simulink model "hrg_bias_tdm_separate"  (R2025a)
settings: Solver=FixedStepDiscrete  StartTime=0.0  StopTime=(floor(c.duration/L.T+1e-9)-1)*L.T  FixedStep=L.T  RelTol=1e-3
model workspace (MAT data in the model file):
  L.F = [0.999580876972 3.24694996317e-07 6.81989764392e-05 6.22779391701e-05 5.91705719226e-22 1.19137426687e-24 -3.75693094649e-06 -6.22765091713e-07 0.0307885035579 6.20769031032e-05 0 0 ... (676 elements, 26x26)]
  L.G = [-0.000337166724513  -2.04304384739e-07  -0.00375589625801  5.33282123475e-09; -2.04543780755e-07  -0.000336718961012  3.19516910592e-09  -0.00375590559772; 0.00375588661538  -2.39457733197e-08  -0.000337166687299  -2.0423130018e-07; -2.18248235755e-08  0.00375593674255  -2.04470629604e-07  -0.000336719083954; 2.59647192694e-23  -2.85679187492e-28  -4.5702926148e-24  -1.40870743879e-27; -7.50589339501e-28  7.17545438659e-23  -3.90090208289e-27  -1.26447354992e-23; -3.75578257448e-05  2.40080747261e-10  3.383220588e-06  2.0422391658e-09; 2.18872587298e-10  -3.75583283826e-05  2.04463898185e-09  3.37874470913e-06; 0.00374197693059  -3.01302631226e-08  -0.000452279130212  -2.03304674872e-07; -2.80246387116e-08  0.00374204062084  -2.03608755041e-07  -0.000451833485601; 0  0  0  0; 0  0  0  0; -0.00154586308247  -1.73922924704e-07  -0.00321638953928  7.06995124769e-08; -1.74820024684e-07  -0.00154548114517  6.88761221884e-08  -0.00321654240012; 0  0  0  0; 0  0  0  0; -0.00236595352656  -1.3071982655e-07  -0.00241196525268  1.1512833246e-07; -1.32042498131e-07  -0.00236566575377  1.13754487179e-07  -0.00241221592121; 0  0  0  0; 0  0  0  0; -0.0028559083186  -7.99186721916e-08  -0.00144095630782  1.42291193957e-07; -8.1478017053e-08  -0.00285573155971  1.414473285e-07  -0.00144126705338; 0  0  0  0; 0  0  0  0; -0.00299916333611  -2.7641740102e-08  -0.000421240643113  1.51686649037e-07; -2.92493876018e-08  -0.00299910102992  1.51389176194e-07  -0.000421572566559]
  L.Hm = [0.999684417191  -1.48369934019e-06  -4.27964442652e-05  -4.66872440298e-05  -8.76929181689e-06  -4.76033457184e-09  -2.77456675998e-15  -3.69759326305e-16  2.43670473864e-11  3.69053916892e-14  0  0  0  0  0  0  0  0  0  0  0  0  0  0  0  0; -9.95250815563e-07  0.999687132089  -4.67001934864e-05  5.94798760013e-05  -4.76590244423e-09  -8.75885884545e-06  -3.69863076005e-16  -1.96454498714e-15  3.69274884564e-14  2.4286186882e-11  0  0  0  0  0  0  0  0  0  0  0  0  0  0  0  0; 7.61663704353e-05  4.67327413513e-05  0.999689714407  3.47258972194e-06  0.000102201297366  -5.08100401249e-11  7.91754167661e-12  2.73891160432e-17  -7.91004583605e-10  -1.61451620118e-15  0  0  0  0  0  0  0  0  0  0  0  0  0  0  0  0; 4.66938598472e-05  -2.61528408374e-05  3.96124178836e-06  0.999681573002  -9.63729064099e-13  0.000102201354068  3.12592084879e-17  7.91747744597e-12  -2.0008486826e-15  -7.91000624119e-10  0  0  0  0  0  0  0  0  0  0  0  0  0  0  0  0]
  L.Jm = [-0.000337106170818  -1.45329445201e-07  -0.00375629387149  4.42303169643e-09; -1.4556259223e-07  -0.000336787590847  2.90233098369e-09  -0.0037563018941; 0.00375629287294  -4.43692118232e-09  -0.000337233307174  -1.47097873108e-07; -2.91469077935e-09  0.0037563009243  -1.47136257932e-07  -0.000336911066999]
  L.Hc = [0.999712525524  1.91858120311e-06  -6.15968747997e-05  -4.30791897988e-05  -8.77146029918e-06  -4.42130011438e-09  -2.92353463991e-15  -3.41191828511e-16  2.43826074769e-11  3.41333263065e-14  0  0  -1.05090176987e-17  0  0  0  -6.61884364746e-19  0  0  0  -2.78073123766e-20  0  0  0  -5.84450076089e-22  0; 2.36910188548e-06  0.999707829722  -4.30567486948e-05  3.27377280262e-05  -4.4229173289e-09  -8.76177426388e-06  -3.41015192585e-16  -2.17639320848e-15  3.41264969975e-14  2.43078504888e-11  0  0  0  -1.05090176987e-17  0  0  0  -6.61884364746e-19  0  0  0  -2.78073123766e-20  0  0  0  -5.84450076089e-22; 6.4439329659e-05  4.41588003056e-05  0.999705540775  2.16132091986e-06  0.000102203018173  -1.62298309029e-10  7.91766705e-12  1.7010139137e-17  -7.91017391745e-10  -6.39624237198e-16  0  0  1.62851688606e-17  0  0  0  1.04154327129e-18  0  0  0  4.44136721082e-20  0  0  0  9.47053371996e-22  0; 4.41337760248e-05  -3.22571857823e-05  2.62312072719e-06  0.999700300936  -1.15318707191e-10  0.000102203322214  2.06675279441e-17  7.91762578606e-12  -1.00437249736e-15  -7.91015591268e-10  0  0  0  1.62851688606e-17  0  0  0  1.04154327129e-18  0  0  0  4.44136721082e-20  0  0  0  9.47053371996e-22]
  L.Jc = [-0.000337186287065  -1.32918322919e-07  -0.0037563931516  -9.57826075507e-09; -1.33005698555e-07  -0.000336895051636  -1.0968370094e-08  -0.00375637064928; 0.00375635629289  -8.4966552311e-09  -0.000337194577217  -1.36983680769e-07; -7.07999835389e-09  0.00375637335218  -1.37065085409e-07  -0.000336894443708]
  L.T = 0.000588235294118
  L.cvMap = [0.1458556769 -1.25015829619e-05 0.150764764274 -1.24845611429e-05 0.155664550533 -1.24667221104e-05 0.160554733441 -1.24480654683e-05 0.165435011352 -1.24285908741e-05 0.170305083231 -1.24082980387e-05 ... (96000 elements, 3200x30)]
  L.candidateOffset_s = 0.000515625
  biasWeights = [2.25592531536e-13; -5.76887878015e-06; 6.31924199918e-06; -0.00170881215954; 0.000155581549194]
  c.mode = 'tdm_separate'
  c.reuse = 0
  c.continuous = 0
  c.Ts = 1.83823529412e-07
  c.w = 42725.6600888
  c.omega = -0.001
  c.duration = 20
  c.B = 0.276990961962
  c.n = 800
  c.adcLatency = 5
  c.logDecimation = 200
  c.p.schema = 'v10.1'
  c.p.synthetic = 1
  c.p.f0 = 6800
  c.p.gamma_intrinsic = 0.712094334814
  c.p.Cs = 7.2e-10
  c.p.G0 = 1e-10
  c.p.kappa = 1e-06
  c.p.b = 1.1e-06
  c.p.Cds = 0
  c.p.Rs = 1000
  c.p.B = 0.276990961962
  c.p.Omega = -0.001
  c.p.Ts = 1.83823529412e-07
  c.p.Tc = 0.001
  c.p.duration = 20
  c.p.charge_target = 1e-11
  c.p.initial_fraction = 1
  c.p.theta0 = 0.981747704247
  c.p.Cf = 1e-10
  c.p.Rf = 1000000000
  c.p.driver_tau = [2e-06; 2e-06]
  c.p.afe_bw = [20000; 20000]
  c.p.detect_matrix = [1  0; 0  1]
  c.p.drive_matrix = [20  0; 0  20]
  c.p.split_hz = 0.05
  c.p.stiffness_axis = 0.37
  c.p.damping_half_difference = 0
  c.p.damping_axis = -0.23
  c.p.adc_span = 2
  c.p.adc_bits = 40
  c.p.dac_span = 1
  c.p.dac_bits = 40
  c.p.vmax = 0.5
  c.p.agc_bw = 10
  c.p.quad_bw = 4
  c.p.pll_gain = 30
  c.p.max_detune = 30
  c.p.virtual_rate = 0
  c.p.virtual_start_min_s = 0.25
  c.p.virtual_settle_fraction = 0.01
  c.p.predict_heading = 1
  c.p.max_heading_rate = 100
  c.p.virtual_validated_limit = 0.2
  c.p.min_amplitude_fraction = 0.02
  c.p.min_linearity = 0.1
  c.p.max_calibration_condition = 100
  c.p.max_frame_age = 0.002
  c.p.calibrate_detection = 1
  c.p.calibrate_drive = 1
  c.p.noise_rms_V = 0
  c.p.noise_seed = 52
  c.p.carrier_hz = 6800
  c.p.Q = 30000
  c.p.pre_gain = 1
  c.p.power_gain = 20
  c.p.aaf_order = 4
  c.p.fs = 5440000
  c.p.bleed_R = 2777.77854938
  c.p.reset_tau = 2e-06
  c.p.adc_latency = 5
  c.p.log_decimation = 200
  c.p.adc_noise_rms = 0
  c.p.adc_dither_lsb_rms = 0
  c.p.adc_dither_seeds = [1103515245; 2246822519]
  c.p.dac_divisor = 1
  c.p.allow_adc_underclock = 0
  c.p.seed_enabled = 0
  c.p.seed_seconds = 0.03
  c.p.seed_voltage = 0.2
  c.p.cv_mode = 'thx2024'
  c.p.thx_cv_gain = 10000
  c.p.thx_charge_per_input = 1e-06
  c.p.cv_source = 'thx2024'
  c.head.f0_Hz = 6800
  c.head.split_Hz = 0.05
  c.head.Q = 30000
  c.head.parasitic_F = 7.2e-10
  c.head.f_modes_Hz = [6799.975 6800.025]
  c.head.ringdown_s = 1.4043083214
  c.head.linewidth_Hz = 0.226666666667
  c.head.temperature_model = 'No per-head temperature curve supplied'
  c.head.group_shunt_F = [7.2e-10; 7.2e-10; 7.2e-10; 7.2e-10]
  c.driveEnd = 800
  c.senseStart = 1200
  c.validStart = 2000
  c.validEnd = 2800
  c.frame = 3200
  c.adcStep = 1.81898940355e-12
  c.adcMin = -1
  c.adcMax = 0.999999999998
  c.dacStep = 9.09494701773e-13
  c.dacMin = -0.5
  c.dacMax = 0.499999999999
  c.minEnergy = 0.0004
  c.minLinearity = 0.1
  c.agc = 62.8318530718
  c.gamma = 0.712094334814
  c.quad = 25.1327412287
  c.forceScale = 3.10732073373
  c.startCommand = [0; 0; 0; 0]
  c.seedCommand = [0; 0; -0.111114046604; -0.166293922461]
  c.stateCount = 26
  c.pickoff = [0  0  0  0  0  0  0  0  0  0  0  0  0  0  0  0  0  0  0  0  0  0  0  0  -0.8  0; 0  0  0  0  0  0  0  0  0  0  0  0  0  0  0  0  0  0  0  0  0  0  0  0  0  -0.8]
  c.motion = [1  0  0  0  0  0  0  0  0  0  0  0  0  0  0  0  0  0  0  0  0  0  0  0  0  0; 0  1  0  0  0  0  0  0  0  0  0  0  0  0  0  0  0  0  0  0  0  0  0  0  0  0]
  c.electrode = [0  0  0  0  0  0  0  0  -0.000427256600888  0  0  0  0  0  0  0  0  0  0  0  0  0  0  0  0  0; 0  0  0  0  0  0  0  0  0  -0.000427256600888  0  0  0  0  0  0  0  0  0  0  0  0  0  0  0  0]
  c.cvOutputGain = 10000
  c.Ad = [0.999969157815 1.52913483819e-10 -0.0078538572151 3.89384302746e-08 -2.77791419972e-24 3.37636119045e-29 7.54624297663e-05 -3.74133744973e-10 -0.000922446324141 4.57342487404e-09 0 0 ... (676 elements, 26x26)]
  c.Bd = [9.92930166753e-10  -3.47455020638e-20; 6.32815022009e-20  9.92930166722e-10; 3.90624565077e-07  -1.63776477948e-17; 3.51196242248e-17  3.90624565057e-07; 0.0878143670381  -3.30600504134e-39; 1.4384601036e-38  0.0878143670381; 3956.34070317  1.48469609002e-19; -3.08984060094e-19  3956.34070317; 3.03749598347e-08  -1.07224009297e-18; 1.96290342016e-18  3.03749598337e-08; 0  0; 0  0; 2.63190636606e-13  -6.89445846608e-24; 1.05402170351e-23  2.63190636602e-13; 0  0; 0  0; 9.85537732628e-16  -2.28470915408e-26; 3.30795441844e-26  9.85537732617e-16; 0  0; 0  0; 3.16265867511e-18  -6.57380608771e-29; 9.12786227069e-29  3.16265867508e-18; 0  0; 0  0; 8.88208109573e-21  -1.67304894509e-31; 2.24711851914e-31  8.88208109567e-21]
  c.Af = [0.999969157815 1.52913483819e-10 -0.0078538572151 3.89384302746e-08 -2.77791419972e-24 3.37636119045e-29 7.54624297663e-05 -3.74133744973e-10 -0.000922446324141 4.57342487404e-09 0 0 ... (676 elements, 26x26)]
  c.As = [0.999969157815 1.52913483819e-10 -0.0078538572151 3.89384302746e-08 -2.77791419972e-24 3.37636119045e-29 7.54624297663e-05 -3.74133744973e-10 -0.000922446324141 4.57342487404e-09 0 0 ... (676 elements, 26x26)]
  c.x0 = [0.55557023302; 0.831469612303; 0; 0; 0; 0; 0; 0; 0; 0; 0; 0; 0; 0; 0; 0; 0; 0; 0; 0; 0; 0; 0; 0; 0; 0]
  c.detect = [-0.353453438315  0  -1.51577588934  0; 0  -0.353453438315  0  -1.51577588934; 1.51577588934  0  -0.353453438315  0; 0  1.51577588934  0  -0.353453438315]
  c.drive = [0.049981589959  0  0.00448426958854  0; 0  0.049981589959  0  0.00448426958854; -0.00448426958854  0  0.049981589959  0; 0  -0.00448426958854  0  0.049981589959]
  c.gain_check.drive_pre_V_per_V = 1
  c.gain_check.sense_pre_V_per_V = 1
  c.gain_check.driver_post_gain = 20
  c.gain_check.detector_V_per_normalized_charge = 0.642491786495
  c.gain_check.electrode_limit_V = 10
  c.gain_check.drive_modal_V_per_command = 19.9273260068
  c.gain_check.drive_condition = 1
  c.gain_check.sense_condition = 1
  c.thx_comparison.saved_Kcvd = 10000
  c.thx_comparison.saved_Kcvs = 100000
  c.thx_comparison.saved_Kcsd = 10000
  c.thx_comparison.saved_Kcss = 100000
  c.thx_comparison.matched_cv_gain = 10000
  c.thx_comparison.piezo_charge_per_input_unit_C = 1e-06
  c.thx_comparison.reuse_scope = 'THX static readout Gain, matched to drive channel source value. Piezo adapter and AAF are external.'
  c.stateRows = {'1:4', '5:6', '7:10', '11:26'}
  c.portDriveMap = [1  0; 0  1; 0  0; 0  0]
  c.portSenseMap = [0  0  -8  0; 0  0  0  -8]
  c.portCoupling = [1  0; 0  1; -1  0; 0  -1]
  c.portCapacitance_F = [7.2e-10  0  0  0; 0  7.2e-10  0  0; 0  0  7.2e-10  0; 0  0  0  7.2e-10]
  c.portShuntCapacitance_F = [7.2e-10; 7.2e-10; 7.2e-10; 7.2e-10]
  c.groupAngles_deg = [0; 45; 90; 135]
  c.groupNames = {'A', 'B', 'C', 'D'}
  c.commonTerminal = 'COM'
  c.portOptions.group_angles_deg = [0; 45; 90; 135]
  c.portOptions.group_charge_gain = [1; 1; 1; 1]
  c.portOptions.group_capacitance_F = [7.2e-10; 7.2e-10; 7.2e-10; 7.2e-10]
  c.portOptions.drive_on_resistance_ohm = 10
  c.portOptions.diagnostic_carrier_phase_rad = []
  c.portCV = [0  0  0  0  0  0  0  0  0  0  0  0  0  0  0  0  0  0  0  0  0  0  0.1  0  0  0; 0  0  0  0  0  0  0  0  0  0  0  0  0  0  0  0  0  0  0  0  0  0  0  0.1  0  0; 0  0  0  0  0  0  0  0  0  0  0  0  0  0  0  0  0  0  0  0  0  0  0  0  0.1  0; 0  0  0  0  0  0  0  0  0  0  0  0  0  0  0  0  0  0  0  0  0  0  0  0  0  0.1]
  c.groupVoltage = [0  0  0  0  0  0  0.000427256600888  0  0  0  0  0  0  0  0  0  0  0  0  0  0  0  0  0  0  0; 0  0  0  0  0  0  0  0.000427256600888  0  0  0  0  0  0  0  0  0  0  0  0  0  0  0  0  0  0; 0  0  0  0  0  0  0  0  0.000427256600888  0  0  0  0  0  0  0  0  0  0  0  0  0  0  0  0  0; 0  0  0  0  0  0  0  0  0  0.000427256600888  0  0  0  0  0  0  0  0  0  0  0  0  0  0  0  0]
  c.periodicCarrier = 1
settings Model: Creator=Administrator  LastModifiedBy=Administrator

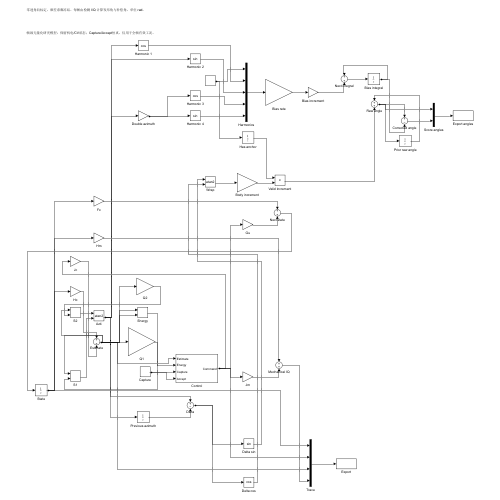
[thumbnail: Simulink's stored preview of the top-level diagram]
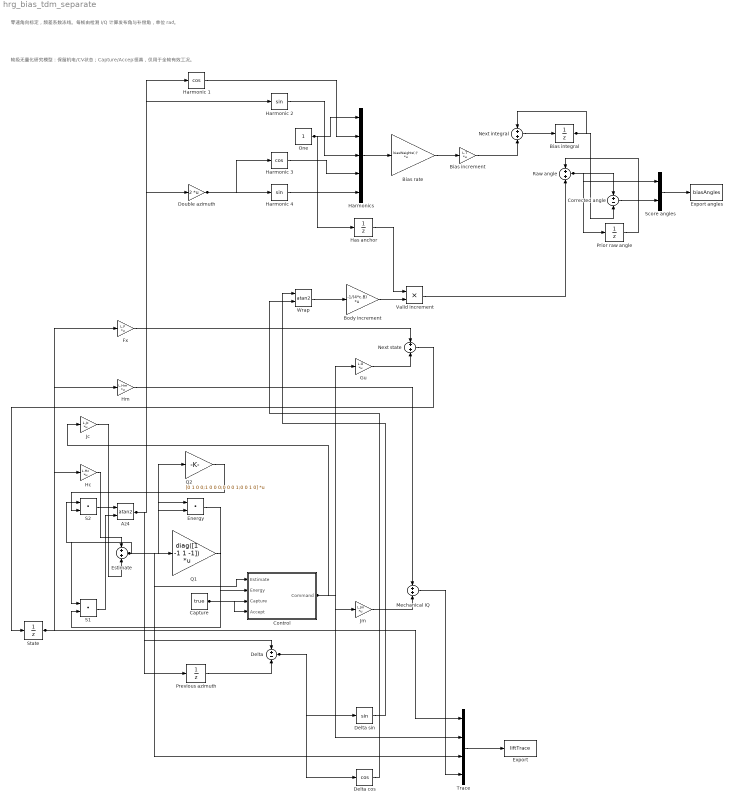
== system hrg_bias_tdm_separate ==
  note: 帧级无量化研究模型：保留机电/CV状态；Capture/Accept恒真，仅用于全帧有效工况。
  note: 零速角向标定，频差系数冻结。每帧由检测 I/Q 计算发布角与补偿角，单位 rad。
  Az4 : Trigonometry  Operator=atan2
  Bias increment : Gain  Gain=L.T  Multiplication=Matrix(K*u)
  Bias integral : UnitDelay  SampleTime=L.T  HasFrameUpgradeWarning=on
  Bias rate : Gain  Gain=biasWeights(:)'  Multiplication=Matrix(K*u)
  Body increment : Gain  Gain=-1/(4*c.B)  Multiplication=Matrix(K*u)
  Capture : Constant  Value=true  OutDataTypeStr=boolean
  Control : Subsystem
  Corrected angle : Sum  Inputs=+-
  Delta : Sum  Inputs=+-
  Delta cos : Trigonometry  Operator=cos
  Delta sin : Trigonometry
  Double azimuth : Gain  Gain=2  Multiplication=Matrix(K*u)
  Energy : DotProduct  OutDataTypeStr=Inherit: Inherit via internal rule
  Estimate : Sum
  Export : ToWorkspace  VariableName=liftTrace  SampleTime=-1
  Export angles : ToWorkspace  VariableName=biasAngles  SampleTime=-1
  Fx : Gain  Gain=L.F  Multiplication=Matrix(K*u)
  Gu : Gain  Gain=L.G  Multiplication=Matrix(K*u)
  Harmonic 1 : Trigonometry  Operator=cos
  Harmonic 2 : Trigonometry
  Harmonic 3 : Trigonometry  Operator=cos
  Harmonic 4 : Trigonometry
  Harmonics : Mux  Inputs=5
  Has anchor : UnitDelay  SampleTime=L.T  HasFrameUpgradeWarning=on
  Hc : Gain  Gain=L.Hc  Multiplication=Matrix(K*u)
  Hm : Gain  Gain=L.Hm  Multiplication=Matrix(K*u)
  Jc : Gain  Gain=L.Jc  Multiplication=Matrix(K*u)
  Jm : Gain  Gain=L.Jm  Multiplication=Matrix(K*u)
  Mechanical IQ : Sum
  Next integral : Sum
  Next state : Sum
  One : Constant
  Previous azimuth : UnitDelay  SampleTime=L.T  HasFrameUpgradeWarning=on
  Prior raw angle : UnitDelay  SampleTime=L.T  HasFrameUpgradeWarning=on
  Q1 : Gain  Gain=diag([1 -1 1 -1])  Multiplication=Matrix(K*u)
  Q2 : Gain  Gain=[0 1 0 0;1 0 0 0;0 0 0 1;0 0 1 0]  Multiplication=Matrix(K*u)
  Raw angle : Sum
  S1 : DotProduct  OutDataTypeStr=Inherit: Inherit via internal rule
  S2 : DotProduct  OutDataTypeStr=Inherit: Inherit via internal rule
  Score angles : Mux  Inputs=2
  State : UnitDelay  InitialCondition=c.x0  SampleTime=-1  HasFrameUpgradeWarning=on
  Trace : Mux
  Valid increment : Product
  Wrap : Trigonometry  Operator=atan2
  wires:
  Score angles/1 -> Export angles/1
  Corrected angle/1 -> Score angles/2
  Control/1(Command) -> Jc/1, Trace/2, Gu/1, Jm/1
  Hm/1 -> Mechanical IQ/1
  Hc/1 -> Estimate/1
  Jc/1 -> Estimate/2
  State/1 -> Fx/1, Hm/1, Hc/1, Trace/1
  S1/1 -> Az4/2
  Az4/1 -> Harmonic 2/1, Double azimuth/1, Harmonic 1/1, Previous azimuth/1, Delta/1
  S2/1 -> Az4/1
  Raw angle/1 -> Corrected angle/1, Score angles/1, Prior raw angle/1
  Energy/1 -> Control/2(Energy)
  Fx/1 -> Next state/1
  Prior raw angle/1 -> Raw angle/1
  Estimate/1 -> Control/1(Estimate), Energy/1, Q1/1, Q2/1, Trace/3, S1/1, Energy/2, S2/1
  Harmonic 1/1 -> Harmonics/2
  Double azimuth/1 -> Harmonic 4/1, Harmonic 3/1
  Q2/1 -> S2/2
  Q1/1 -> S1/2
  Capture/1 -> Control/4(Accept), Control/3(Capture)
  Wrap/1 -> Body increment/1
  Previous azimuth/1 -> Delta/2
  Bias rate/1 -> Bias increment/1
  Harmonic 2/1 -> Harmonics/3
  Harmonics/1 -> Bias rate/1
  One/1 -> Harmonics/1, Has anchor/1
  Harmonic 3/1 -> Harmonics/4
  Harmonic 4/1 -> Harmonics/5
  Delta cos/1 -> Wrap/2
  Delta/1 -> Delta sin/1, Delta cos/1
  Has anchor/1 -> Valid increment/1
  Body increment/1 -> Valid increment/2
  Mechanical IQ/1 -> Trace/4
  Gu/1 -> Next state/2
  Next state/1 -> State/1
  Jm/1 -> Mechanical IQ/2
  Bias integral/1 -> Next integral/1, Corrected angle/2
  Next integral/1 -> Bias integral/1
  Delta sin/1 -> Wrap/1
  Valid increment/1 -> Raw angle/2
  Bias increment/1 -> Next integral/2
  Trace/1 -> Export/1

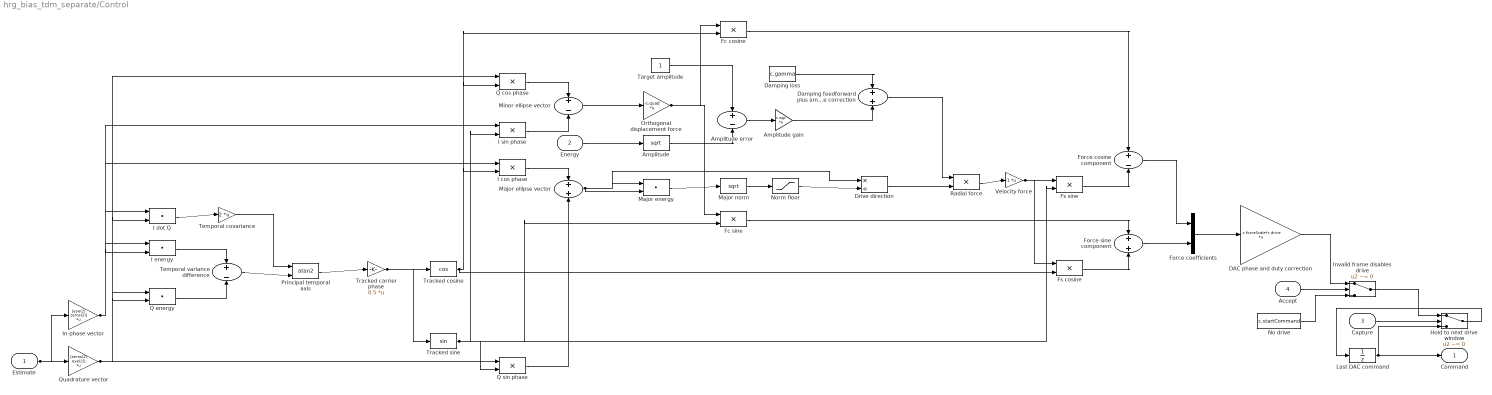
== system hrg_bias_tdm_separate/Control ==
  Estimate : Inport
  Energy : Inport  Port=2
  Capture : Inport  Port=3
  Accept : Inport  Port=4
  Amplitude : Sqrt
  Amplitude error : Sum  Inputs=+-
  Amplitude gain : Gain  Gain=c.agc  Multiplication=Matrix(K*u)
  DAC phase and duty correction : Gain  Gain=c.forceScale*c.drive  Multiplication=Matrix(K*u)
  Damping feedforward plus amplitude correction : Sum
  Damping loss : Constant  Value=c.gamma
  Drive direction : Product  Inputs=*/
  Fc cosine : Product
  Fc sine : Product
  Force coefficients : Mux  Inputs=2
  Force cosine component : Sum  Inputs=+-
  Force sine component : Sum
  Fs cosine : Product
  Fs sine : Product
  Hold to next drive window : Switch  Criteria=u2 ~= 0  SaturateOnIntegerOverflow=off  InputSameDT=off
  I cos phase : Product
  I dot Q : DotProduct  OutDataTypeStr=Inherit: Inherit via internal rule
  I energy : DotProduct  OutDataTypeStr=Inherit: Inherit via internal rule
  I sin phase : Product
  In-phase vector : Gain  Gain=[eye(2) zeros(2)]  Multiplication=Matrix(K*u)
  Invalid frame disables drive : Switch  Criteria=u2 ~= 0  SaturateOnIntegerOverflow=off  InputSameDT=off
  Last DAC command : UnitDelay  InitialCondition=c.startCommand  SampleTime=L.T  HasFrameUpgradeWarning=on
  Major ellipse vector : Sum
  Major energy : DotProduct  OutDataTypeStr=Inherit: Inherit via internal rule
  Major norm : Sqrt
  Minor ellipse vector : Sum  Inputs=+-
  No drive : Constant  Value=c.startCommand
  Norm floor : Saturate  UpperLimit=inf  LowerLimit=1e-9
  Orthogonal displacement force : Gain  Gain=-c.quad  Multiplication=Matrix(K*u)
  Principal temporal axis : Trigonometry  Operator=atan2
  Q cos phase : Product
  Q energy : DotProduct  OutDataTypeStr=Inherit: Inherit via internal rule
  Q sin phase : Product
  Quadrature vector : Gain  Gain=[zeros(2) eye(2)]  Multiplication=Matrix(K*u)
  Radial force : Product
  Target amplitude : Constant
  Temporal covariance : Gain  Gain=2  Multiplication=Matrix(K*u)
  Temporal variance difference : Sum  Inputs=+-
  Tracked carrier phase : Gain  Gain=0.5  Multiplication=Matrix(K*u)
  Tracked cosine : Trigonometry  Operator=cos
  Tracked sine : Trigonometry
  Velocity force : Gain  Gain=-1  Multiplication=Matrix(K*u)
  Command : Outport
  wires:
  Last DAC command/1 -> Hold to next drive window/3, Command/1
  No drive/1 -> Invalid frame disables drive/3
  Accept/1 -> Invalid frame disables drive/2
  DAC phase and duty correction/1 -> Invalid frame disables drive/1
  Force coefficients/1 -> DAC phase and duty correction/1
  Fs cosine/1 -> Force sine component/2
  Drive direction/1 -> Radial force/2
  Damping feedforward plus amplitude correction/1 -> Radial force/1
  Norm floor/1 -> Drive direction/2
  Amplitude gain/1 -> Damping feedforward plus amplitude correction/2
  Force cosine component/1 -> Force coefficients/1
  Damping loss/1 -> Damping feedforward plus amplitude correction/1
  Capture/1 -> Hold to next drive window/2
  Major norm/1 -> Norm floor/1
  Major energy/1 -> Major norm/1
  Amplitude/1 -> Amplitude error/2
  Orthogonal displacement force/1 -> Fc cosine/1, Fc sine/1
  Target amplitude/1 -> Amplitude error/1
  Amplitude error/1 -> Amplitude gain/1
  Major ellipse vector/1 -> Major energy/2, Major energy/1, Drive direction/1
  Energy/1 -> Amplitude/1
  Force sine component/1 -> Force coefficients/2
  Minor ellipse vector/1 -> Orthogonal displacement force/1
  Velocity force/1 -> Fs cosine/1, Fs sine/1
  Q sin phase/1 -> Major ellipse vector/2
  I sin phase/1 -> Minor ellipse vector/2
  Fc cosine/1 -> Force cosine component/1
  Q cos phase/1 -> Minor ellipse vector/1
  I cos phase/1 -> Major ellipse vector/1
  Invalid frame disables drive/1 -> Hold to next drive window/1
  Tracked sine/1 -> I sin phase/2, Q sin phase/2, Fc sine/2, Fs sine/2
  Hold to next drive window/1 -> Last DAC command/1
  Tracked cosine/1 -> Fs cosine/2, Q cos phase/2, I cos phase/2, Fc cosine/2
  Fc sine/1 -> Force sine component/1
  Tracked carrier phase/1 -> Tracked sine/1, Tracked cosine/1
  Q energy/1 -> Temporal variance difference/2
  I energy/1 -> Temporal variance difference/1
  Fs sine/1 -> Force cosine component/2
  Quadrature vector/1 -> Q energy/1, Q energy/2, I dot Q/2, Q cos phase/1, Q sin phase/1
  Principal temporal axis/1 -> Tracked carrier phase/1
  Temporal covariance/1 -> Principal temporal axis/1
  Temporal variance difference/1 -> Principal temporal axis/2
  Estimate/1 -> Quadrature vector/1, In-phase vector/1
  In-phase vector/1 -> I cos phase/1, I sin phase/1, I dot Q/1, I energy/1, I energy/2
  I dot Q/1 -> Temporal covariance/1
  Radial force/1 -> Velocity force/1
